simulink model "A21_S6504193_Martinenghi"  (R2026a)
settings: Solver=ode15s  MaxStep=1e-3  RelTol=1e-4
PreLoadFcn:
  | a21_init_robot
values from neighbouring files (symbols this model uses):
  corner_base = 0.15    [a21_init_robot.m]
  g_0 = bRw * g'    [a21_init_robot.m]
  I = zeros(3, 3, n_links)    [a21_init_robot.m]
  len = [lenght_l1, lenght_l2, lenght_l3]    [a21_init_robot.m]
  lenght_cyl = 0.07    [a21_init_robot.m]
  lenght_l1 = 0.2    [a21_init_robot.m]
  lenght_l2 = 0.2    [a21_init_robot.m]
  lenght_l3 = 0.2    [a21_init_robot.m]
  mass = [mass_l1, mass_l2, mass_l3]    [a21_init_robot.m]
  mass_ee = 0    [a21_init_robot.m]
  mass_joint = 0    [a21_init_robot.m]
  mass_l1 = 2.5    [a21_init_robot.m]
  mass_l2 = 4.5    [a21_init_robot.m]
  mass_l3 = 1.5    [a21_init_robot.m]
  q1_f = deg2rad(60)    [a21_init_robot.m]
  q1_i = deg2rad(20)    [a21_init_robot.m]
  q2_f = deg2rad(-15)    [a21_init_robot.m]
  q2_i = deg2rad(30)    [a21_init_robot.m]
  q3_f = deg2rad(40)    [a21_init_robot.m]
  q3_i = deg2rad(-10)    [a21_init_robot.m]
  width = 0.01    [a21_init_robot.m]
undefined symbols (not defined in the file or in its folder): X, Y, Z
libraries: nesl_utility x35, sm_lib x28, robotcorelib x3, simulink x3
settings Model: Creator=ubuntu  LastModifiedBy=ubuntu

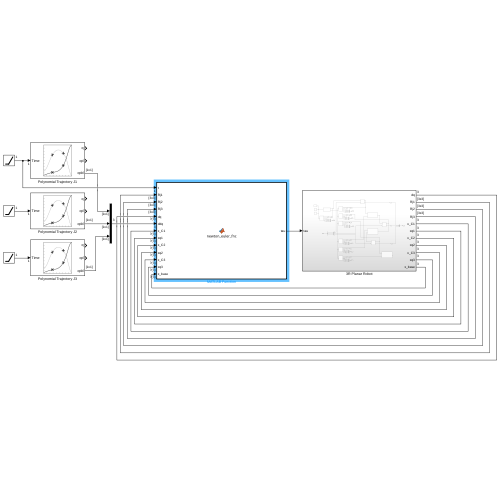
[thumbnail: Simulink's stored preview of the top-level diagram]
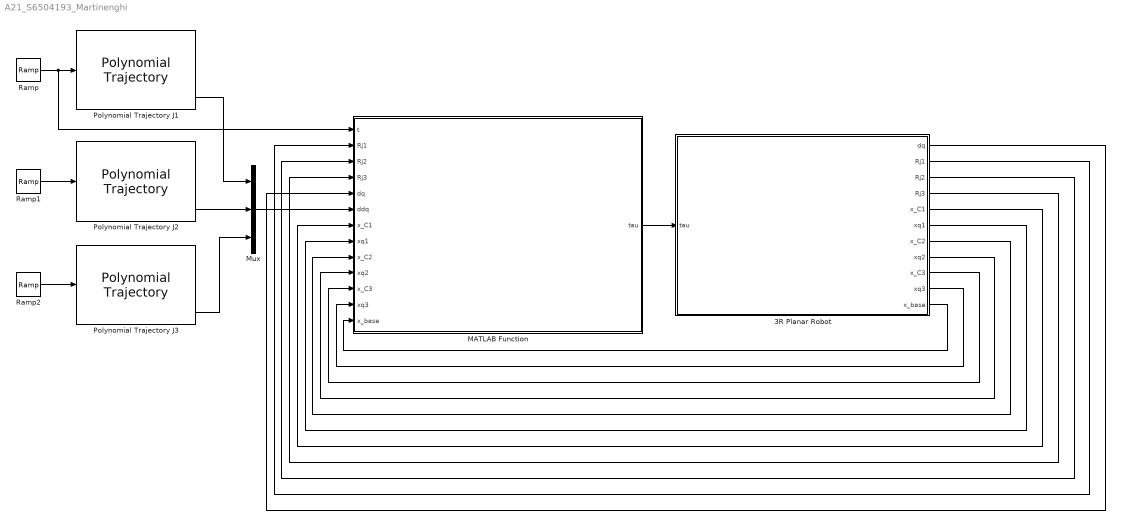
== system A21_S6504193_Martinenghi ==
  3R Planar Robot : Subsystem
  MATLAB Function : MATLAB Function  TreatAsAtomicUnit=on
  Mux : Mux  Inputs=3
  Polynomial Trajectory J1 : robotcorelib/Polynomial Trajectory  WaypointSource=Internal  Waypoints=[q1_i, q1_f]  TimePoints=[ 0, 10 ]  TimeInterval=[ 1, 4 ]  Method=Cubic Polynomial  ParameterSource=Internal  VelocityBoundaryCondition=zeros( 1, 2 )  AccelerationBoundaryCondition=zeros( 2, 5 )  SimulateUsing=Interpreted execution
  Polynomial Trajectory J2 : robotcorelib/Polynomial Trajectory  WaypointSource=Internal  Waypoints=[ q2_i, q2_f ]  TimePoints=[ 0, 10 ]  TimeInterval=[ 1, 4 ]  Method=Cubic Polynomial  ParameterSource=Internal  VelocityBoundaryCondition=zeros( 1, 2 )  AccelerationBoundaryCondition=zeros( 2, 5 )  SimulateUsing=Interpreted execution
  Polynomial Trajectory J3 : robotcorelib/Polynomial Trajectory  WaypointSource=Internal  Waypoints=[ q3_i, q3_f ]  TimePoints=[ 0, 10 ]  TimeInterval=[ 1, 4 ]  Method=Cubic Polynomial  ParameterSource=Internal  VelocityBoundaryCondition=zeros( 1, 2 )  AccelerationBoundaryCondition=zeros( 2, 5 )  SimulateUsing=Interpreted execution
  Ramp : simulink/Sources/Ramp  slope=1  start=0  InitialOutput=0
  Ramp1 : simulink/Sources/Ramp  slope=1  start=0  InitialOutput=0
  Ramp2 : simulink/Sources/Ramp  slope=1  start=0  InitialOutput=0
  wires:
  MATLAB Function/1(tau) -> 3R Planar Robot/1(tau)
  Ramp/1 -> MATLAB Function/1(t), Polynomial Trajectory J1/1
  Ramp1/1 -> Polynomial Trajectory J2/1
  Polynomial Trajectory J1/3 -> Mux/1
  Polynomial Trajectory J2/3 -> Mux/2
  Ramp2/1 -> Polynomial Trajectory J3/1
  Polynomial Trajectory J3/3 -> Mux/3
  Mux/1 -> MATLAB Function/6(ddq)
  3R Planar Robot/1(dq) -> MATLAB Function/5(dq)
  3R Planar Robot/2(Rj1) -> MATLAB Function/2(Rj1)
  3R Planar Robot/3(Rj2) -> MATLAB Function/3(Rj2)
  3R Planar Robot/4(Rj3) -> MATLAB Function/4(Rj3)
  3R Planar Robot/5(x_C1) -> MATLAB Function/7(x_C1)
  3R Planar Robot/6(xq1) -> MATLAB Function/8(xq1)
  3R Planar Robot/7(x_C2) -> MATLAB Function/9(x_C2)
  3R Planar Robot/8(xq2) -> MATLAB Function/10(xq2)
  3R Planar Robot/9(x_C3) -> MATLAB Function/11(x_C3)
  3R Planar Robot/10(xq3) -> MATLAB Function/12(xq3)
  3R Planar Robot/11(x_base) -> MATLAB Function/13(x_base)

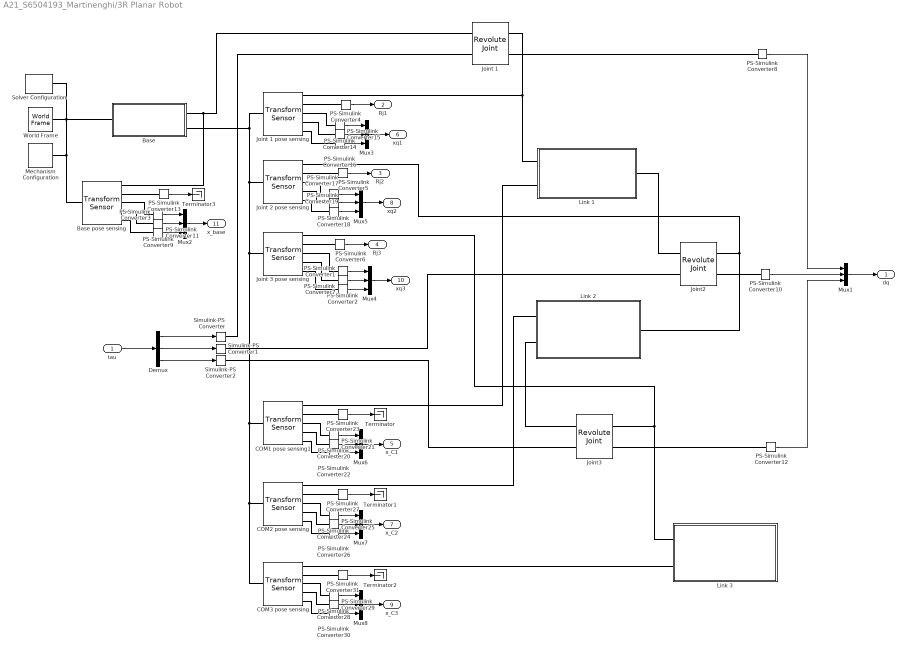
== system A21_S6504193_Martinenghi/3R Planar Robot ==
  tau : Inport  Unit=1
  Base : Subsystem
      settings: PortSchema="{\"entries\":[{\"content\":{\"sides\":[{\"content\":{},\"type\":\"ConnectorPlacement.EquallySpacedRectSide\",\"uuid\":\"d02f94b6-e832-47a0-a34b-6833663c7bb5\"},{\"content\":{\"side\":\"RIGHT\"},\"type\":\"ConnectorPlacement.EquallySpacedRectSide\",\"uuid\":\"6125681a-8698-4101-8864-7244487dafa4\"},{\"content\":{\"connectorIds\":[\"LConn1\"],\"side\":\"TOP\"},\"type\":\"ConnectorPlacement.EquallySpacedRectSide\",\"uuid\":\"6c8db9f7-c5c0-485a-b6d5-359a8a80284c\"},{\"content\":{\"connectorIds\":[\"RConn1\",\"RConn2\"],\"side\":\"BOTTOM\"},\"type\":\"ConnectorPlacement.EquallySpacedRectSide\",\"uuid\":\"97f1219d-93fc-432b-9e6b-1b8efba6c947\"}]},\"type\":\"ConnectorPlacement.EquallySpacedConnector\",\"uuid\":\"ff6e16aa-4c4e-4070-a58f-244657740585\"}],\"packageUris\":[\"http://schema.mathworks.com/mf0/Connector/R2020b\"],\"version\":\"1.0\"}"
  Base pose sensing : sm_lib/Frames and Transforms/Transform Sensor  MeasurementFrame=Base  RotationSequence=XYX  SenseAngle=off  SenseAxis=off  SenseQ=off  SenseR=on  SenseRotationSequence=off  SenseOmegaX=off  SenseOmegaY=off  SenseOmegaZ=off  SenseOmega=off  SenseQDot=off  SenseRDot=off  SenseRotationSequenceDot=off  SenseAlphaX=off  SenseAlphaY=off  SenseAlphaZ=off  SenseAlpha=off  SenseQDDot=off  SenseRDDot=off  SenseX=on  SenseY=on  SenseZ=on  SenseXYZ=off  SenseRad=off  SenseAzim=off  SenseDist=off  SenseInc=off  SenseXDot=off  SenseYDot=off  SenseZDot=off  SenseXYZDot=off  SenseRadDot=off  SenseAzimDot=off  SenseDistDot=off  SenseIncDot=off  SenseXDDot=off  SenseYDDot=off  SenseZDDot=off  SenseXYZDDot=off  SenseRadDDot=off  SenseAzimDDot=off  SenseDistDDot=off  SenseIncDDot=off
  COM1 pose sensing1 : sm_lib/Frames and Transforms/Transform Sensor  MeasurementFrame=Base  RotationSequence=XYX  SenseAngle=off  SenseAxis=off  SenseQ=off  SenseR=on  SenseRotationSequence=off  SenseOmegaX=off  SenseOmegaY=off  SenseOmegaZ=off  SenseOmega=off  SenseQDot=off  SenseRDot=off  SenseRotationSequenceDot=off  SenseAlphaX=off  SenseAlphaY=off  SenseAlphaZ=off  SenseAlpha=off  SenseQDDot=off  SenseRDDot=off  SenseX=on  SenseY=on  SenseZ=on  SenseXYZ=off  SenseRad=off  SenseAzim=off  SenseDist=off  SenseInc=off  SenseXDot=off  SenseYDot=off  SenseZDot=off  SenseXYZDot=off  SenseRadDot=off  SenseAzimDot=off  SenseDistDot=off  SenseIncDot=off  SenseXDDot=off  SenseYDDot=off  SenseZDDot=off  SenseXYZDDot=off  SenseRadDDot=off  SenseAzimDDot=off  SenseDistDDot=off  SenseIncDDot=off
  COM2 pose sensing : sm_lib/Frames and Transforms/Transform Sensor  MeasurementFrame=Base  RotationSequence=XYX  SenseAngle=off  SenseAxis=off  SenseQ=off  SenseR=on  SenseRotationSequence=off  SenseOmegaX=off  SenseOmegaY=off  SenseOmegaZ=off  SenseOmega=off  SenseQDot=off  SenseRDot=off  SenseRotationSequenceDot=off  SenseAlphaX=off  SenseAlphaY=off  SenseAlphaZ=off  SenseAlpha=off  SenseQDDot=off  SenseRDDot=off  SenseX=on  SenseY=on  SenseZ=on  SenseXYZ=off  SenseRad=off  SenseAzim=off  SenseDist=off  SenseInc=off  SenseXDot=off  SenseYDot=off  SenseZDot=off  SenseXYZDot=off  SenseRadDot=off  SenseAzimDot=off  SenseDistDot=off  SenseIncDot=off  SenseXDDot=off  SenseYDDot=off  SenseZDDot=off  SenseXYZDDot=off  SenseRadDDot=off  SenseAzimDDot=off  SenseDistDDot=off  SenseIncDDot=off
  COM3 pose sensing : sm_lib/Frames and Transforms/Transform Sensor  MeasurementFrame=Base  RotationSequence=XYX  SenseAngle=off  SenseAxis=off  SenseQ=off  SenseR=on  SenseRotationSequence=off  SenseOmegaX=off  SenseOmegaY=off  SenseOmegaZ=off  SenseOmega=off  SenseQDot=off  SenseRDot=off  SenseRotationSequenceDot=off  SenseAlphaX=off  SenseAlphaY=off  SenseAlphaZ=off  SenseAlpha=off  SenseQDDot=off  SenseRDDot=off  SenseX=on  SenseY=on  SenseZ=on  SenseXYZ=off  SenseRad=off  SenseAzim=off  SenseDist=off  SenseInc=off  SenseXDot=off  SenseYDot=off  SenseZDot=off  SenseXYZDot=off  SenseRadDot=off  SenseAzimDot=off  SenseDistDot=off  SenseIncDot=off  SenseXDDot=off  SenseYDDot=off  SenseZDDot=off  SenseXYZDDot=off  SenseRadDDot=off  SenseAzimDDot=off  SenseDistDDot=off  SenseIncDDot=off
  Demux : Demux  Outputs=3
  Joint 1 : sm_lib/Joints/Revolute Joint  JointMode=Normal  CompositeWrenchDir=FollowerOnBase  CompositeWrenchFrame=BaseFrame  SenseConstraintForce=off  SenseConstraintTorque=off  SenseTotalForce=off  SenseTotalTorque=off  PositionTargetSpecify=on  PositionTargetPriority=High  PositionTargetValue=q1_i  PositionTargetValueUnits=rad  VelocityTargetSpecify=off  VelocityTargetPriority=High  VelocityTargetValue=0  VelocityTargetValueUnits=deg/s  EquilibriumPosition=0  EquilibriumPositionUnits=deg  SpringStiffness=0  SpringStiffnessUnits=N*m/deg  DampingCoefficient=0  DampingCoefficientUnits=N*m/(deg/s)  LowerLimitSpecify=off  LowerLimitBound=-90  LowerLimitBoundUnits=deg  LowerLimitStiffness=1e4  LowerLimitStiffnessUnits=N*m/deg  LowerLimitDamping=10  LowerLimitDampingUnits=N*m/(deg/s)  LowerLimitTransitionRegionWidth=0.1  LowerLimitTransitionRegionWidthUnits=deg  UpperLimitSpecify=off  UpperLimitBound=90  UpperLimitBoundUnits=deg  UpperLimitStiffness=1e4  UpperLimitStiffnessUnits=N*m/deg  UpperLimitDamping=10  UpperLimitDampingUnits=N*m/(deg/s)  UpperLimitTransitionRegionWidth=0.1  UpperLimitTransitionRegionWidthUnits=deg  TorqueActuationMode=InputTorque  MotionActuationMode=ComputedMotion  SensePosition=off  SenseVelocity=on  SenseAcceleration=off  SenseTorqueForce=off  SenseLowerLimitTorqueForce=off  SenseUpperLimitTorqueForce=off
  Joint 1 pose sensing : sm_lib/Frames and Transforms/Transform Sensor  MeasurementFrame=Base  RotationSequence=XYX  SenseAngle=off  SenseAxis=off  SenseQ=off  SenseR=on  SenseRotationSequence=off  SenseOmegaX=off  SenseOmegaY=off  SenseOmegaZ=off  SenseOmega=off  SenseQDot=off  SenseRDot=off  SenseRotationSequenceDot=off  SenseAlphaX=off  SenseAlphaY=off  SenseAlphaZ=off  SenseAlpha=off  SenseQDDot=off  SenseRDDot=off  SenseX=on  SenseY=on  SenseZ=on  SenseXYZ=off  SenseRad=off  SenseAzim=off  SenseDist=off  SenseInc=off  SenseXDot=off  SenseYDot=off  SenseZDot=off  SenseXYZDot=off  SenseRadDot=off  SenseAzimDot=off  SenseDistDot=off  SenseIncDot=off  SenseXDDot=off  SenseYDDot=off  SenseZDDot=off  SenseXYZDDot=off  SenseRadDDot=off  SenseAzimDDot=off  SenseDistDDot=off  SenseIncDDot=off
  Joint 2 pose sensing : sm_lib/Frames and Transforms/Transform Sensor  MeasurementFrame=Base  RotationSequence=XYX  SenseAngle=off  SenseAxis=off  SenseQ=off  SenseR=on  SenseRotationSequence=off  SenseOmegaX=off  SenseOmegaY=off  SenseOmegaZ=off  SenseOmega=off  SenseQDot=off  SenseRDot=off  SenseRotationSequenceDot=off  SenseAlphaX=off  SenseAlphaY=off  SenseAlphaZ=off  SenseAlpha=off  SenseQDDot=off  SenseRDDot=off  SenseX=on  SenseY=on  SenseZ=on  SenseXYZ=off  SenseRad=off  SenseAzim=off  SenseDist=off  SenseInc=off  SenseXDot=off  SenseYDot=off  SenseZDot=off  SenseXYZDot=off  SenseRadDot=off  SenseAzimDot=off  SenseDistDot=off  SenseIncDot=off  SenseXDDot=off  SenseYDDot=off  SenseZDDot=off  SenseXYZDDot=off  SenseRadDDot=off  SenseAzimDDot=off  SenseDistDDot=off  SenseIncDDot=off
  Joint 3 pose sensing : sm_lib/Frames and Transforms/Transform Sensor  MeasurementFrame=Base  RotationSequence=XYX  SenseAngle=off  SenseAxis=off  SenseQ=off  SenseR=on  SenseRotationSequence=off  SenseOmegaX=off  SenseOmegaY=off  SenseOmegaZ=off  SenseOmega=off  SenseQDot=off  SenseRDot=off  SenseRotationSequenceDot=off  SenseAlphaX=off  SenseAlphaY=off  SenseAlphaZ=off  SenseAlpha=off  SenseQDDot=off  SenseRDDot=off  SenseX=on  SenseY=on  SenseZ=on  SenseXYZ=off  SenseRad=off  SenseAzim=off  SenseDist=off  SenseInc=off  SenseXDot=off  SenseYDot=off  SenseZDot=off  SenseXYZDot=off  SenseRadDot=off  SenseAzimDot=off  SenseDistDot=off  SenseIncDot=off  SenseXDDot=off  SenseYDDot=off  SenseZDDot=off  SenseXYZDDot=off  SenseRadDDot=off  SenseAzimDDot=off  SenseDistDDot=off  SenseIncDDot=off
  Joint2 : sm_lib/Joints/Revolute Joint  JointMode=Normal  CompositeWrenchDir=FollowerOnBase  CompositeWrenchFrame=BaseFrame  SenseConstraintForce=off  SenseConstraintTorque=off  SenseTotalForce=off  SenseTotalTorque=off  PositionTargetSpecify=on  PositionTargetPriority=High  PositionTargetValue=q2_i  PositionTargetValueUnits=rad  VelocityTargetSpecify=off  VelocityTargetPriority=High  VelocityTargetValue=0  VelocityTargetValueUnits=deg/s  EquilibriumPosition=0  EquilibriumPositionUnits=deg  SpringStiffness=0  SpringStiffnessUnits=N*m/deg  DampingCoefficient=0  DampingCoefficientUnits=N*m/(deg/s)  LowerLimitSpecify=off  LowerLimitBound=-90  LowerLimitBoundUnits=deg  LowerLimitStiffness=1e4  LowerLimitStiffnessUnits=N*m/deg  LowerLimitDamping=10  LowerLimitDampingUnits=N*m/(deg/s)  LowerLimitTransitionRegionWidth=0.1  LowerLimitTransitionRegionWidthUnits=deg  UpperLimitSpecify=off  UpperLimitBound=90  UpperLimitBoundUnits=deg  UpperLimitStiffness=1e4  UpperLimitStiffnessUnits=N*m/deg  UpperLimitDamping=10  UpperLimitDampingUnits=N*m/(deg/s)  UpperLimitTransitionRegionWidth=0.1  UpperLimitTransitionRegionWidthUnits=deg  TorqueActuationMode=InputTorque  MotionActuationMode=ComputedMotion  SensePosition=off  SenseVelocity=on  SenseAcceleration=off  SenseTorqueForce=off  SenseLowerLimitTorqueForce=off  SenseUpperLimitTorqueForce=off
  Joint3 : sm_lib/Joints/Revolute Joint  JointMode=Normal  CompositeWrenchDir=FollowerOnBase  CompositeWrenchFrame=BaseFrame  SenseConstraintForce=off  SenseConstraintTorque=off  SenseTotalForce=off  SenseTotalTorque=off  PositionTargetSpecify=on  PositionTargetPriority=High  PositionTargetValue=q3_i  PositionTargetValueUnits=rad  VelocityTargetSpecify=off  VelocityTargetPriority=High  VelocityTargetValue=0  VelocityTargetValueUnits=deg/s  EquilibriumPosition=0  EquilibriumPositionUnits=deg  SpringStiffness=0  SpringStiffnessUnits=N*m/deg  DampingCoefficient=0  DampingCoefficientUnits=N*m/(deg/s)  LowerLimitSpecify=off  LowerLimitBound=-90  LowerLimitBoundUnits=deg  LowerLimitStiffness=1e4  LowerLimitStiffnessUnits=N*m/deg  LowerLimitDamping=10  LowerLimitDampingUnits=N*m/(deg/s)  LowerLimitTransitionRegionWidth=0.1  LowerLimitTransitionRegionWidthUnits=deg  UpperLimitSpecify=off  UpperLimitBound=90  UpperLimitBoundUnits=deg  UpperLimitStiffness=1e4  UpperLimitStiffnessUnits=N*m/deg  UpperLimitDamping=10  UpperLimitDampingUnits=N*m/(deg/s)  UpperLimitTransitionRegionWidth=0.1  UpperLimitTransitionRegionWidthUnits=deg  TorqueActuationMode=InputTorque  MotionActuationMode=ComputedMotion  SensePosition=off  SenseVelocity=on  SenseAcceleration=off  SenseTorqueForce=off  SenseLowerLimitTorqueForce=off  SenseUpperLimitTorqueForce=off
  Link 1 : Subsystem
      settings: PortSchema="{\"entries\":[{\"content\":{\"sides\":[{\"content\":{},\"type\":\"ConnectorPlacement.EquallySpacedRectSide\",\"uuid\":\"e8e71268-e230-47e9-97b7-0270bcf34c4f\"},{\"content\":{\"side\":\"RIGHT\"},\"type\":\"ConnectorPlacement.EquallySpacedRectSide\",\"uuid\":\"ce6cc1b2-c4ca-4a44-a462-c641e93c28d9\"},{\"content\":{\"connectorIds\":[\"LConn1\",\"LConn2\"],\"side\":\"TOP\"},\"type\":\"ConnectorPlacement.EquallySpacedRectSide\",\"uuid\":\"d1ee8f4a-9d35-43b6-b82c-c9cfc2349581\"},{\"content\":{\"connectorIds\":[\"RConn1\"],\"side\":\"BOTTOM\"},\"type\":\"ConnectorPlacement.EquallySpacedRectSide\",\"uuid\":\"35d9e855-2c2a-487f-8a8c-86808fcf10bc\"}]},\"type\":\"ConnectorPlacement.EquallySpacedConnector\",\"uuid\":\"9066da4f-4459-4153-a610-9898f54d88e7\"}],\"packageUris\":[\"http://schema.mathworks.com/mf0/Connector/R2020b\"],\"version\":\"1.0\"}"
  Link 2 : Subsystem
  Link 3 : Subsystem
  Mechanism Configuration : sm_lib/Utilities/Mechanism Configuration  UniformGravity=Constant  GravityVector=g  GravityVectorUnits=m/s^2  LinearizationDelta=0.001  JointModeTransitionNonlinearIterations=2
  Mux{1..8} (8 alike) : Mux  Inputs=3
  PS-Simulink Converter{1..31} (31 alike) : nesl_utility/PS-Simulink Converter  PhysicalDomain=network_engine_domain  SubClassName=ps_output  LeftPortType=input  RightPortType=output  PseudoPeriodic=off  Frequencies=[]  VectorFormat=inherit  Unit=inherit  AffineConversion=off
  Simulink-PS Converter : nesl_utility/Simulink-PS Converter  PhysicalDomain=network_engine_domain  SubClassName=ps_input  LeftPortType=input  RightPortType=output  PseudoPeriodic=off  Frequencies=[]  NoiseDistribution=none  NoiseParameters=[]  Unit=1  AffineConversion=off  FilteringAndDerivatives=provide  SimscapeFilterOrder=1  InputFilterTimeConstant=0.001  UdotUserProvided=0
  Simulink-PS Converter1 : nesl_utility/Simulink-PS Converter  PhysicalDomain=network_engine_domain  SubClassName=ps_input  LeftPortType=input  RightPortType=output  PseudoPeriodic=off  Frequencies=[]  NoiseDistribution=none  NoiseParameters=[]  Unit=1  AffineConversion=off  FilteringAndDerivatives=provide  SimscapeFilterOrder=1  InputFilterTimeConstant=0.001  UdotUserProvided=0
  Simulink-PS Converter2 : nesl_utility/Simulink-PS Converter  PhysicalDomain=network_engine_domain  SubClassName=ps_input  LeftPortType=input  RightPortType=output  PseudoPeriodic=off  Frequencies=[]  NoiseDistribution=none  NoiseParameters=[]  Unit=1  AffineConversion=off  FilteringAndDerivatives=provide  SimscapeFilterOrder=1  InputFilterTimeConstant=0.001  UdotUserProvided=0
  Solver Configuration : nesl_utility/Solver Configuration  PhysicalDomain=network_engine_domain  SubClassName=solver  LeftPortType=input  RightPortType=generic  Tones=[]  Harmonics=[]  SimulateNoise=off  Profile=off  UseLocalSampling=off  EnableSwitchedLinearOptims=on  FrequencyDomain=off  UseCCode=off  RelTol=0.001  AbsTol=0.001  MinStep=1e-09  ToWorkspace=off  RevertToSquareIcSolve=off  NumHomotopyIterations=100  PhasorMode=off  PhasorModeNumHarmonics=1  ConsistencySolver=NEWTON_XTOL_AFTER_FTOL  CanonicalOrdering=CANONICAL  OptimizeIntermediates=OPTIMIZED  IndexReductionMethod=DerivativeReplacement  DoDC=off  ResidualTolerance=1e-09  ConsistencyTolSource=GLOBAL  ConsistencyAbsTol=0.001  ConsistencyRelTol=0.001  ConsistencyTolFactor=0.001  UseLocalSolver=off  LocalSolverChoice=NE_BACKWARD_EULER_ADVANCER  ResolveIndetEquations=on  FunctionEvalNumThread=1  LocalSolverSampleTime=0.001  DoFixedCost=off  MaxNonlinIter=3  MaxModeIter=2  ComputeImpulses=off  ImpulseIterations=2  LinearAlgebra=auto  LinearAlgebraNumThread=0  EquationFormulation=NE_TIME_EF  DelaysMemoryBudget=1024  AutomaticFiltering=on  FilteringTimeConstant=0.001  PartitionStorageMethod=AS_NEEDED  PartitionMemoryBudget=1024  PartitionMethod=ROBUST  MultibodyUseLocalSolver=off  MultibodyLocalSolverChoice=ODE1  MultibodyLocalSolverSampleTime=0.001
  Terminator{,1..3} (4 alike) : Terminator
  World Frame : sm_lib/Frames and Transforms/World Frame
  dq : Outport
  Rj1 : Outport  Port=2
  Rj2 : Outport  Port=3
  Rj3 : Outport  Port=4
  x_C1 : Outport  Port=5
  xq1 : Outport  Port=6
  x_C2 : Outport  Port=7
  xq2 : Outport  Port=8
  x_C3 : Outport  Port=9
  xq3 : Outport  Port=10
  x_base : Outport  Port=11
  wires:
  tau/1 -> Demux/1
  PS-Simulink Converter8/1 -> Mux1/1
  PS-Simulink Converter10/1 -> Mux1/2
  PS-Simulink Converter5/1 -> Rj2/1
  PS-Simulink Converter4/1 -> Rj1/1
  Demux/1 -> Simulink-PS Converter/1
  PS-Simulink Converter12/1 -> Mux1/3
  Demux/2 -> Simulink-PS Converter1/1
  Mux1/1 -> dq/1
  Demux/3 -> Simulink-PS Converter2/1
  PS-Simulink Converter6/1 -> Rj3/1
  PS-Simulink Converter15/1 -> Mux3/2
  PS-Simulink Converter14/1 -> Mux3/1
  PS-Simulink Converter16/1 -> Mux3/3
  Mux3/1 -> xq1/1
  PS-Simulink Converter2/1 -> Mux4/2
  PS-Simulink Converter1/1 -> Mux4/1
  Mux4/1 -> xq3/1
  PS-Simulink Converter7/1 -> Mux4/3
  PS-Simulink Converter18/1 -> Mux5/2
  PS-Simulink Converter17/1 -> Mux5/1
  Mux5/1 -> xq2/1
  PS-Simulink Converter19/1 -> Mux5/3
  PS-Simulink Converter23/1 -> Terminator/1
  PS-Simulink Converter22/1 -> Mux6/3
  Mux6/1 -> x_C1/1
  PS-Simulink Converter21/1 -> Mux6/2
  PS-Simulink Converter20/1 -> Mux6/1
  PS-Simulink Converter26/1 -> Mux7/3
  Mux7/1 -> x_C2/1
  PS-Simulink Converter24/1 -> Mux7/1
  PS-Simulink Converter25/1 -> Mux7/2
  PS-Simulink Converter27/1 -> Terminator1/1
  PS-Simulink Converter30/1 -> Mux8/3
  Mux8/1 -> x_C3/1
  PS-Simulink Converter28/1 -> Mux8/1
  PS-Simulink Converter29/1 -> Mux8/2
  PS-Simulink Converter31/1 -> Terminator2/1
  PS-Simulink Converter9/1 -> Mux2/2
  PS-Simulink Converter3/1 -> Mux2/1
  Mux2/1 -> x_base/1
  PS-Simulink Converter13/1 -> Terminator3/1
  PS-Simulink Converter11/1 -> Mux2/3
  connections:
  Link 1/RConn1 -- Joint2/LConn1
  Simulink-PS Converter/RConn1 -- Joint 1/LConn2
  PS-Simulink Converter12/LConn1 -- Joint3/RConn2
  Joint3/RConn1 -- Joint 3 pose sensing/RConn1 -- Link 3/LConn1
  Link 2/RConn2 -- Joint3/LConn1
  Joint2/RConn1 -- Joint 2 pose sensing/RConn1 -- Link 2/LConn1
  Base/RConn2 -- Base pose sensing/RConn1 -- Joint 1/LConn1
  Joint 1/RConn1 -- Joint 1 pose sensing/RConn1 -- Link 1/LConn1
  PS-Simulink Converter4/LConn1 -- Joint 1 pose sensing/RConn2
  PS-Simulink Converter8/LConn1 -- Joint 1/RConn2
  Simulink-PS Converter2/RConn1 -- Joint3/LConn2
  PS-Simulink Converter5/LConn1 -- Joint 2 pose sensing/RConn2
  Simulink-PS Converter1/RConn1 -- Joint2/LConn2
  PS-Simulink Converter6/LConn1 -- Joint 3 pose sensing/RConn2
  World Frame/RConn1 -- Mechanism Configuration/RConn1 -- Base pose sensing/LConn1 -- Base/LConn1 -- Solver Configuration/RConn1
  Base/RConn1 -- Joint 1 pose sensing/LConn1 -- COM3 pose sensing/LConn1 -- COM2 pose sensing/LConn1 -- COM1 pose sensing1/LConn1 -- Joint 3 pose sensing/LConn1 -- Joint 2 pose sensing/LConn1
  Joint 1 pose sensing/RConn3 -- PS-Simulink Converter14/LConn1
  Joint 1 pose sensing/RConn5 -- PS-Simulink Converter16/LConn1
  Joint 1 pose sensing/RConn4 -- PS-Simulink Converter15/LConn1
  PS-Simulink Converter1/LConn1 -- Joint 3 pose sensing/RConn3
  PS-Simulink Converter7/LConn1 -- Joint 3 pose sensing/RConn5
  PS-Simulink Converter2/LConn1 -- Joint 3 pose sensing/RConn4
  Joint 2 pose sensing/RConn3 -- PS-Simulink Converter17/LConn1
  Joint 2 pose sensing/RConn5 -- PS-Simulink Converter19/LConn1
  Joint 2 pose sensing/RConn4 -- PS-Simulink Converter18/LConn1
  COM1 pose sensing1/RConn5 -- PS-Simulink Converter22/LConn1
  COM1 pose sensing1/RConn4 -- PS-Simulink Converter21/LConn1
  COM1 pose sensing1/RConn3 -- PS-Simulink Converter20/LConn1
  PS-Simulink Converter23/LConn1 -- COM1 pose sensing1/RConn2
  COM2 pose sensing/RConn5 -- PS-Simulink Converter26/LConn1
  COM2 pose sensing/RConn3 -- PS-Simulink Converter24/LConn1
  COM2 pose sensing/RConn4 -- PS-Simulink Converter25/LConn1
  PS-Simulink Converter27/LConn1 -- COM2 pose sensing/RConn2
  COM3 pose sensing/RConn5 -- PS-Simulink Converter30/LConn1
  COM3 pose sensing/RConn3 -- PS-Simulink Converter28/LConn1
  COM3 pose sensing/RConn4 -- PS-Simulink Converter29/LConn1
  PS-Simulink Converter31/LConn1 -- COM3 pose sensing/RConn2
  Link 1/LConn2 -- COM1 pose sensing1/RConn1
  Link 2/RConn1 -- COM2 pose sensing/RConn1
  Link 3/LConn2 -- COM3 pose sensing/RConn1
  Joint2/RConn2 -- PS-Simulink Converter10/LConn1
  Base pose sensing/RConn4 -- PS-Simulink Converter9/LConn1
  PS-Simulink Converter13/LConn1 -- Base pose sensing/RConn2
  Base pose sensing/RConn5 -- PS-Simulink Converter11/LConn1
  Base pose sensing/RConn3 -- PS-Simulink Converter3/LConn1

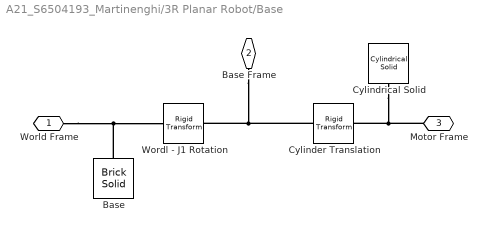
== system A21_S6504193_Martinenghi/3R Planar Robot/Base ==
  Base : sm_lib/Body Elements/Brick Solid  BrickDimensions=[corner_base width corner_base]  BrickDimensionsUnits=m  ExportEntireGeometry=off  InertiaType=CalculateFromGeometry  BasedOnType=Mass  Density=1000  DensityUnits=kg/m^3  Mass=mass_joint  MassUnits=kg  CenterOfMass=[0 0 0]  CenterOfMassUnits=m  MomentsOfInertia=[1 1 1]  MomentsOfInertiaUnits=kg*m^2  ProductsOfInertia=[0 0 0]  ProductsOfInertiaUnits=kg*m^2  GraphicType=FromGeometry  MarkerShape=Sphere  MarkerSize=10  GraphicVisPropType=SimpleVisualProperties  GraphicDiffuseColor=[0.5 0.5 0.5]  GraphicOpacity=1  GraphicSpecularColor=[0.5 0.5 0.5 1.0]  GraphicAmbientColor=[0.15 0.15 0.15 1.0]  GraphicEmissiveColor=[0.0 0.0 0.0 1.0]  GraphicShininess=75  DoExposeReferenceFrame=on  SerializedFrames=<Frames/>
  Cylinder Translation : sm_lib/Frames and Transforms/Rigid Transform  RotationMethod=None  FollAlignAxisA=+X  BaseAlignAxisA=+Y  FollAlignAxisB=+Y  BaseAlignAxisB=+Z  RotationStandardAxis=+X  RotationAngle=-90  RotationAngleUnits=deg  RotationArbitraryAxis=[0 0 1]  RotationSequenceAxes=FollowerAxes  RotationSequence=XYX  RotationSequenceAngles=[0 0 0]  RotationSequenceAnglesUnits=deg  RotationMatrix=[1 0 0;0 1 0;0 0 1]  Quaternion=[1 0 0 0]  TranslationMethod=StandardAxis  TranslationCartesianOffset=[0 0 0]  TranslationCartesianOffsetUnits=m  TranslationStandardAxis=+Z  TranslationStandardOffset=lenght_cyl/2  TranslationStandardOffsetUnits=m  TranslationROffset=0  TranslationROffsetUnits=m  TranslationThetaOffset=0  TranslationThetaOffsetUnits=deg  TranslationZOffset=0  TranslationZOffsetUnits=m
  Cylindrical Solid : sm_lib/Body Elements/Cylindrical Solid  CylinderRadius=radius_cyl  CylinderRadiusUnits=m  CylinderLength=lenght_cyl  CylinderLengthUnits=m  ExportEntireGeometry=off  InertiaType=CalculateFromGeometry  BasedOnType=Mass  Density=1000  DensityUnits=kg/m^3  Mass=mass_joint  MassUnits=kg  CenterOfMass=[0 0 0]  CenterOfMassUnits=m  MomentsOfInertia=[1 1 1]  MomentsOfInertiaUnits=kg*m^2  ProductsOfInertia=[0 0 0]  ProductsOfInertiaUnits=kg*m^2  GraphicType=FromGeometry  MarkerShape=Sphere  MarkerSize=10  GraphicVisPropType=SimpleVisualProperties  GraphicDiffuseColor=[0 0 0]  GraphicOpacity=1  GraphicSpecularColor=[0.5 0.5 0.5 1.0]  GraphicAmbientColor=[0.15 0.15 0.15 1.0]  GraphicEmissiveColor=[0.0 0.0 0.0 1.0]  GraphicShininess=75  DoExposeReferenceFrame=on  SerializedFrames=<Frames/>
  Wordl - J1 Rotation : sm_lib/Frames and Transforms/Rigid Transform  RotationMethod=RotationMatrix  FollAlignAxisA=+X  BaseAlignAxisA=+Y  FollAlignAxisB=+Y  BaseAlignAxisB=+Z  RotationStandardAxis=+X  RotationAngle=90  RotationAngleUnits=deg  RotationArbitraryAxis=[0 0 1]  RotationSequenceAxes=FollowerAxes  RotationSequence=XYX  RotationSequenceAngles=[0 0 0]  RotationSequenceAnglesUnits=deg  RotationMatrix=bRw  Quaternion=[1 0 0 0]  TranslationMethod=None  TranslationCartesianOffset=[0 0 0]  TranslationCartesianOffsetUnits=m  TranslationStandardAxis=+Y  TranslationStandardOffset=-lenght_cyl/2  TranslationStandardOffsetUnits=cm  TranslationROffset=0  TranslationROffsetUnits=m  TranslationThetaOffset=0  TranslationThetaOffsetUnits=deg  TranslationZOffset=0  TranslationZOffsetUnits=m
  World Frame : PMIOPort  Side=Left
  Base Frame : PMIOPort  Port=2  Side=Right
  Motor Frame : PMIOPort  Port=3  Side=Right
  connections:
  World Frame/RConn1 -- Base/RConn1 -- Wordl - J1 Rotation/LConn1
  Cylinder Translation/LConn1 -- Base Frame/RConn1 -- Wordl - J1 Rotation/RConn1
  Motor Frame/RConn1 -- Cylindrical Solid/RConn1 -- Cylinder Translation/RConn1

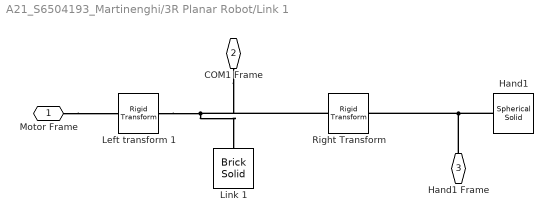
== system A21_S6504193_Martinenghi/3R Planar Robot/Link 1 ==
  Hand1 : sm_lib/Body Elements/Spherical Solid  SphereRadius=radius_sphere  SphereRadiusUnits=m  ExportEntireGeometry=off  InertiaType=CalculateFromGeometry  BasedOnType=Mass  Density=1000  DensityUnits=kg/m^3  Mass=mass_joint  MassUnits=kg  CenterOfMass=[0 0 0]  CenterOfMassUnits=m  MomentsOfInertia=[1 1 1]  MomentsOfInertiaUnits=kg*m^2  ProductsOfInertia=[0 0 0]  ProductsOfInertiaUnits=kg*m^2  GraphicType=FromGeometry  MarkerShape=Sphere  MarkerSize=10  GraphicVisPropType=SimpleVisualProperties  GraphicDiffuseColor=[1 0.7 0]  GraphicOpacity=1  GraphicSpecularColor=[0.5 0.5 0.5 1.0]  GraphicAmbientColor=[0.15 0.15 0.15 1.0]  GraphicEmissiveColor=[0.0 0.0 0.0 1.0]  GraphicShininess=75  DoExposeReferenceFrame=on  SerializedFrames=<Frames/>
  Left transform 1 : sm_lib/Frames and Transforms/Rigid Transform  RotationMethod=None  FollAlignAxisA=+X  BaseAlignAxisA=+Y  FollAlignAxisB=+Y  BaseAlignAxisB=+Z  RotationStandardAxis=+X  RotationAngle=-90  RotationAngleUnits=deg  RotationArbitraryAxis=[0 0 1]  RotationSequenceAxes=FollowerAxes  RotationSequence=XYX  RotationSequenceAngles=[0 0 0]  RotationSequenceAnglesUnits=deg  RotationMatrix=[1 0 0;0 1 0;0 0 1]  Quaternion=[1 0 0 0]  TranslationMethod=StandardAxis  TranslationCartesianOffset=[0 0 0]  TranslationCartesianOffsetUnits=m  TranslationStandardAxis=+X  TranslationStandardOffset=lenght_l1/2  TranslationStandardOffsetUnits=m  TranslationROffset=0  TranslationROffsetUnits=m  TranslationThetaOffset=0  TranslationThetaOffsetUnits=deg  TranslationZOffset=0  TranslationZOffsetUnits=m
  Link 1 : sm_lib/Body Elements/Brick Solid  BrickDimensions=[lenght_l1 width width]  BrickDimensionsUnits=m  ExportEntireGeometry=off  InertiaType=CalculateFromGeometry  BasedOnType=Mass  Density=1000  DensityUnits=kg/m^3  Mass=mass_l1  MassUnits=kg  CenterOfMass=[0 0 0]  CenterOfMassUnits=m  MomentsOfInertia=[1 1 1]  MomentsOfInertiaUnits=kg*m^2  ProductsOfInertia=[0 0 0]  ProductsOfInertiaUnits=kg*m^2  GraphicType=FromGeometry  MarkerShape=Sphere  MarkerSize=10  GraphicVisPropType=SimpleVisualProperties  GraphicDiffuseColor=[0.5 0.5 0.5]  GraphicOpacity=1  GraphicSpecularColor=[0.5 0.5 0.5 1.0]  GraphicAmbientColor=[0.15 0.15 0.15 1.0]  GraphicEmissiveColor=[0.0 0.0 0.0 1.0]  GraphicShininess=75  DoExposeReferenceFrame=on  SerializedFrames=<Frames/>
  Right Transform : sm_lib/Frames and Transforms/Rigid Transform  RotationMethod=None  FollAlignAxisA=+X  BaseAlignAxisA=+Y  FollAlignAxisB=+Y  BaseAlignAxisB=+Z  RotationStandardAxis=+X  RotationAngle=-90  RotationAngleUnits=deg  RotationArbitraryAxis=[0 0 1]  RotationSequenceAxes=FollowerAxes  RotationSequence=ZXZ  RotationSequenceAngles=[-90 -90 0]  RotationSequenceAnglesUnits=deg  RotationMatrix=j1_R_j2  Quaternion=[1 0 0 0]  TranslationMethod=StandardAxis  TranslationCartesianOffset=[0 0 0]  TranslationCartesianOffsetUnits=m  TranslationStandardAxis=+X  TranslationStandardOffset=lenght_l1/2  TranslationStandardOffsetUnits=m  TranslationROffset=0  TranslationROffsetUnits=m  TranslationThetaOffset=0  TranslationThetaOffsetUnits=deg  TranslationZOffset=0  TranslationZOffsetUnits=m
  Motor Frame : PMIOPort  Side=Left
  COM1 Frame : PMIOPort  Port=2  Side=Left
  Hand1 Frame : PMIOPort  Port=3  Side=Right
  connections:
  Left transform 1/RConn1 -- COM1 Frame/RConn1 -- Right Transform/LConn1 -- Link 1/RConn1
  Motor Frame/RConn1 -- Left transform 1/LConn1
  Hand1/RConn1 -- Hand1 Frame/RConn1 -- Right Transform/RConn1

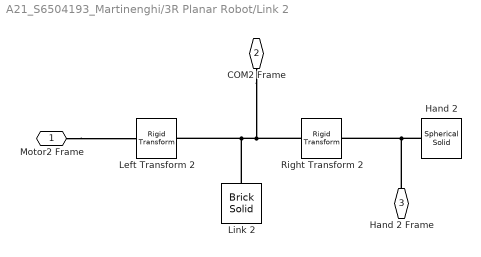
== system A21_S6504193_Martinenghi/3R Planar Robot/Link 2 ==
  Hand 2 : sm_lib/Body Elements/Spherical Solid  SphereRadius=radius_sphere  SphereRadiusUnits=m  ExportEntireGeometry=off  InertiaType=CalculateFromGeometry  BasedOnType=Mass  Density=1000  DensityUnits=kg/m^3  Mass=mass_joint  MassUnits=kg  CenterOfMass=[0 0 0]  CenterOfMassUnits=m  MomentsOfInertia=[1 1 1]  MomentsOfInertiaUnits=kg*m^2  ProductsOfInertia=[0 0 0]  ProductsOfInertiaUnits=kg*m^2  GraphicType=FromGeometry  MarkerShape=Sphere  MarkerSize=10  GraphicVisPropType=SimpleVisualProperties  GraphicDiffuseColor=[1 0.7 0]  GraphicOpacity=1  GraphicSpecularColor=[0.5 0.5 0.5 1.0]  GraphicAmbientColor=[0.15 0.15 0.15 1.0]  GraphicEmissiveColor=[0.0 0.0 0.0 1.0]  GraphicShininess=75  DoExposeReferenceFrame=on  SerializedFrames=<Frames/>
  Left Transform 2 : sm_lib/Frames and Transforms/Rigid Transform  RotationMethod=None  FollAlignAxisA=+X  BaseAlignAxisA=+Y  FollAlignAxisB=+Y  BaseAlignAxisB=+Z  RotationStandardAxis=+Z  RotationAngle=0  RotationAngleUnits=deg  RotationArbitraryAxis=[0 0 1]  RotationSequenceAxes=FollowerAxes  RotationSequence=XYX  RotationSequenceAngles=[0 0 0]  RotationSequenceAnglesUnits=deg  RotationMatrix=[1 0 0;0 1 0;0 0 1]  Quaternion=[1 0 0 0]  TranslationMethod=StandardAxis  TranslationCartesianOffset=[0 0 0]  TranslationCartesianOffsetUnits=m  TranslationStandardAxis=+X  TranslationStandardOffset=lenght_l2/2  TranslationStandardOffsetUnits=m  TranslationROffset=0  TranslationROffsetUnits=m  TranslationThetaOffset=0  TranslationThetaOffsetUnits=deg  TranslationZOffset=0  TranslationZOffsetUnits=m
  Link 2 : sm_lib/Body Elements/Brick Solid  BrickDimensions=[lenght_l2 width width]  BrickDimensionsUnits=m  ExportEntireGeometry=off  InertiaType=CalculateFromGeometry  BasedOnType=Mass  Density=1000  DensityUnits=kg/m^3  Mass=mass_l2  MassUnits=kg  CenterOfMass=[0 0 0]  CenterOfMassUnits=m  MomentsOfInertia=[1 1 1]  MomentsOfInertiaUnits=kg*m^2  ProductsOfInertia=[0 0 0]  ProductsOfInertiaUnits=kg*m^2  GraphicType=FromGeometry  MarkerShape=Sphere  MarkerSize=10  GraphicVisPropType=SimpleVisualProperties  GraphicDiffuseColor=[0.5 0.5 0.5]  GraphicOpacity=1  GraphicSpecularColor=[0.5 0.5 0.5 1.0]  GraphicAmbientColor=[0.15 0.15 0.15 1.0]  GraphicEmissiveColor=[0.0 0.0 0.0 1.0]  GraphicShininess=75  DoExposeReferenceFrame=on  SerializedFrames=<Frames/>
  Right Transform 2 : sm_lib/Frames and Transforms/Rigid Transform  RotationMethod=None  FollAlignAxisA=+X  BaseAlignAxisA=+Y  FollAlignAxisB=+Y  BaseAlignAxisB=+Z  RotationStandardAxis=+Z  RotationAngle=0  RotationAngleUnits=deg  RotationArbitraryAxis=[0 0 1]  RotationSequenceAxes=FollowerAxes  RotationSequence=XYX  RotationSequenceAngles=[0 0 0]  RotationSequenceAnglesUnits=deg  RotationMatrix=[1 0 0;0 1 0;0 0 1]  Quaternion=[1 0 0 0]  TranslationMethod=StandardAxis  TranslationCartesianOffset=[0 0 0]  TranslationCartesianOffsetUnits=m  TranslationStandardAxis=+X  TranslationStandardOffset=lenght_l2/2  TranslationStandardOffsetUnits=m  TranslationROffset=0  TranslationROffsetUnits=m  TranslationThetaOffset=0  TranslationThetaOffsetUnits=deg  TranslationZOffset=0  TranslationZOffsetUnits=m
  Motor2 Frame : PMIOPort  Side=Left
  COM2 Frame : PMIOPort  Port=2  Side=Right
  Hand 2 Frame : PMIOPort  Port=3  Side=Right
  connections:
  Hand 2/RConn1 -- Hand 2 Frame/RConn1 -- Right Transform 2/RConn1
  Motor2 Frame/RConn1 -- Left Transform 2/LConn1
  Right Transform 2/LConn1 -- COM2 Frame/RConn1 -- Left Transform 2/RConn1 -- Link 2/RConn1

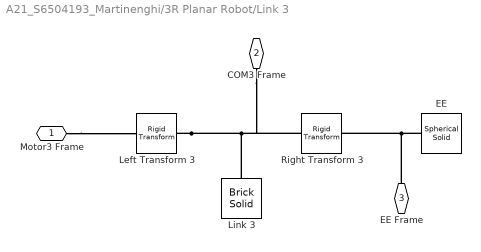
== system A21_S6504193_Martinenghi/3R Planar Robot/Link 3 ==
  EE : sm_lib/Body Elements/Spherical Solid  SphereRadius=radius_sphere  SphereRadiusUnits=m  ExportEntireGeometry=off  InertiaType=CalculateFromGeometry  BasedOnType=Mass  Density=1000  DensityUnits=kg/m^3  Mass=mass_ee  MassUnits=kg  CenterOfMass=[0 0 0]  CenterOfMassUnits=m  MomentsOfInertia=[1 1 1]  MomentsOfInertiaUnits=kg*m^2  ProductsOfInertia=[0 0 0]  ProductsOfInertiaUnits=kg*m^2  GraphicType=FromGeometry  MarkerShape=Sphere  MarkerSize=10  GraphicVisPropType=SimpleVisualProperties  GraphicDiffuseColor=[1 0.7 0]  GraphicOpacity=1  GraphicSpecularColor=[0.5 0.5 0.5 1.0]  GraphicAmbientColor=[0.15 0.15 0.15 1.0]  GraphicEmissiveColor=[0.0 0.0 0.0 1.0]  GraphicShininess=75  DoExposeReferenceFrame=on  SerializedFrames=<Frames/>
  Left Transform 3 : sm_lib/Frames and Transforms/Rigid Transform  RotationMethod=None  FollAlignAxisA=+X  BaseAlignAxisA=+Y  FollAlignAxisB=+Y  BaseAlignAxisB=+Z  RotationStandardAxis=+Z  RotationAngle=0  RotationAngleUnits=deg  RotationArbitraryAxis=[0 0 1]  RotationSequenceAxes=FollowerAxes  RotationSequence=XYX  RotationSequenceAngles=[0 0 0]  RotationSequenceAnglesUnits=deg  RotationMatrix=[1 0 0;0 1 0;0 0 1]  Quaternion=[1 0 0 0]  TranslationMethod=StandardAxis  TranslationCartesianOffset=[0 0 0]  TranslationCartesianOffsetUnits=m  TranslationStandardAxis=+X  TranslationStandardOffset=lenght_l3/2  TranslationStandardOffsetUnits=m  TranslationROffset=0  TranslationROffsetUnits=m  TranslationThetaOffset=0  TranslationThetaOffsetUnits=deg  TranslationZOffset=0  TranslationZOffsetUnits=m
  Link 3 : sm_lib/Body Elements/Brick Solid  BrickDimensions=[lenght_l3 width width]  BrickDimensionsUnits=m  ExportEntireGeometry=off  InertiaType=CalculateFromGeometry  BasedOnType=Mass  Density=1000  DensityUnits=kg/m^3  Mass=mass_l3  MassUnits=kg  CenterOfMass=[0 0 0]  CenterOfMassUnits=m  MomentsOfInertia=[1 1 1]  MomentsOfInertiaUnits=kg*m^2  ProductsOfInertia=[0 0 0]  ProductsOfInertiaUnits=kg*m^2  GraphicType=FromGeometry  MarkerShape=Sphere  MarkerSize=10  GraphicVisPropType=SimpleVisualProperties  GraphicDiffuseColor=[0.5 0.5 0.5]  GraphicOpacity=1  GraphicSpecularColor=[0.5 0.5 0.5 1.0]  GraphicAmbientColor=[0.15 0.15 0.15 1.0]  GraphicEmissiveColor=[0.0 0.0 0.0 1.0]  GraphicShininess=75  DoExposeReferenceFrame=on  SerializedFrames=<Frames/>
  Right Transform 3 : sm_lib/Frames and Transforms/Rigid Transform  RotationMethod=None  FollAlignAxisA=+X  BaseAlignAxisA=+Y  FollAlignAxisB=+Y  BaseAlignAxisB=+Z  RotationStandardAxis=+Z  RotationAngle=0  RotationAngleUnits=deg  RotationArbitraryAxis=[0 0 1]  RotationSequenceAxes=FollowerAxes  RotationSequence=XYX  RotationSequenceAngles=[0 0 0]  RotationSequenceAnglesUnits=deg  RotationMatrix=[1 0 0;0 1 0;0 0 1]  Quaternion=[1 0 0 0]  TranslationMethod=StandardAxis  TranslationCartesianOffset=[0 0 0]  TranslationCartesianOffsetUnits=m  TranslationStandardAxis=+X  TranslationStandardOffset=lenght_l3/2  TranslationStandardOffsetUnits=m  TranslationROffset=0  TranslationROffsetUnits=m  TranslationThetaOffset=0  TranslationThetaOffsetUnits=deg  TranslationZOffset=0  TranslationZOffsetUnits=m
  Motor3 Frame : PMIOPort  Side=Left
  COM3 Frame : PMIOPort  Port=2  Side=Left
  EE Frame : PMIOPort  Port=3  Side=Right
  connections:
  EE/RConn1 -- EE Frame/RConn1 -- Right Transform 3/RConn1
  Motor3 Frame/RConn1 -- Left Transform 3/LConn1
  Left Transform 3/RConn1 -- COM3 Frame/RConn1 -- Right Transform 3/LConn1 -- Link 3/RConn1

== matlab function A21_S6504193_Martinenghi/MATLAB Function ==
  data: t input; Rj1 input; Rj2 input; Rj3 input; dq input; ddq input; g_0 parameter; mass parameter; len parameter; x_C1 input; tau output; xq1 input; x_C2 input; xq2 input; x_C3 input; xq3 input; x_base input; I parameter
function tau = newton_euler_fnc(t, Rj1, Rj2, Rj3, dq, ddq, g_0, mass, len, x_C1, xq1, x_C2, xq2, x_C3, xq3, x_base, I)
    % Rotation matrices from frame i-1 to frame i
    n_links = 3;
    R = zeros(3,3, n_links+1);
    R(:,:,1) = Rj1';          % 0→1
    R(:,:,2) = Rj2' * Rj1;   % 1→2
    R(:,:,3) = Rj3' * Rj2;   % 2→3
    R(:,:,n_links+1) = eye(3); % ee

    Z = [0; 0; 1];

    %% COM positions expressed in frame i (from joint i origin to COM i)
    bx_C = zeros(3, n_links);
    bx_C(:,1) = Rj1' * (x_C1 - xq1);
    bx_C(:,2) = Rj2' * (x_C2 - xq2);
    bx_C(:,3) = Rj3' * (x_C3 - xq3);

    %% Joint-to-joint vectors expressed in frame i-1
    % P(:,i) = vector from joint i-1 to joint i, expressed in frame i-1
    P = zeros(3, n_links+1);
    P(:,1) = x_base;   % base → joint 1
    P(:,2) = [len(1); 0; 0]; % joint 1 → joint 2
    P(:,3) = [len(2); 0; 0]; % joint 2 → joint 3
    P(:,4) = [len(3); 0; 0];      % joint 3 → end-effector

    %% Forward recursion
    omega  = zeros(3, n_links);   % angular velocity
    domega = zeros(3, n_links);   % angular acceleration
    dv     = zeros(3, n_links);   % linear acceleration of joint origin
    dv_C   = zeros(3, n_links);   % linear acceleration of COM
    F      = zeros(3, n_links);   % inertial forces on COMs
    N      = zeros(3, n_links);   % inertial torques on COMs

    for i = 1:n_links
        if i == 1
            omega_prev  = [0; 0; 0];
            domega_prev = [0; 0; 0];
            dv_prev     =  g_0;   % gravity enters here (not negated, not rotated)
        else
            omega_prev  = omega(:, i-1);
            domega_prev = domega(:, i-1);
            dv_prev     = dv(:, i-1);
        end
        
        omega(:,i) = R(:,:,i) * omega_prev + dq(i) * Z; % angular velocity

        domega(:,i) = R(:,:,i) * domega_prev ...
                    + cross(R(:,:,i) * omega_prev, dq(i) * Z) ...
                    + ddq(i) * Z; % angular acceleration

        dv(:,i) = R(:,:,i) * (cross(domega_prev, P(:,i)) ...
                + cross(omega_prev, cross(omega_prev, P(:,i))) ...
                + dv_prev); % linear acceleration of joint i origin

        dv_C(:,i) = cross(domega(:,i), bx_C(:,i)) ...
                  + cross(omega(:,i), cross(omega(:,i), bx_C(:,i))) ...
                  + dv(:,i); % linear acceleration of COM i

        % Inertial force and torque (Newton-Euler)
        F(:,i) = mass(i) * dv_C(:,i);
        N(:,i) = I(:,:,i) * domega(:,i) + cross(omega(:,i), I(:,:,i) * omega(:,i));
    end

    %% Backward recursion
    f   = zeros(3, n_links+1);  % reaction forces
    n   = zeros(3, n_links+1);  % reaction torques
    tau = zeros(n_links, 1);    % output joint torques

    for i = n_links:-1:1
        f(:,i) = R(:,:,i+1)' * f(:,i+1) + F(:,i); % force at joint i

        n(:,i) = N(:,i) ...
               + R(:,:,i+1)' * n(:,i+1) ...
               + cross(bx_C(:,i),   F(:,i)) ...
               + cross(P(:,i+1),   R(:,:,i+1)' * f(:,i+1)); % torque at joint i

        tau(i) = n(:,i)' * Z; % project torque onto joint Z-axis
    end

    if t == 10
        disp("tau1 = ");
        disp(tau(1));
        disp("tau2 = ");
        disp(tau(2));
        disp("tau3 = ");
        disp(tau(3));
    end
end
